simulink library "sfRobotExampleLib"  (R2025b)
settings: Solver=VariableStepAuto  StartTime=0.0  StopTime=10.0  RelTol=1e-3
undefined symbols (not defined in the file or in its folder): boxes, circles, dock
settings Model: Creator=The MathWorks, Inc.  LastModifiedBy=The MathWorks, Inc.
settings OptimizationCC: ReuseModelBlockBuffer=off
settings DebuggingCC: UnconnectedInputMsg=warning  UnconnectedOutputMsg=warning  UnconnectedLineMsg=warning
settings ModelReferenceCC: EnableRefExpFcnMdlSchedulingChecks=on
settings RTWCC: GPUComputeCapability=3.5  DLArmComputeVersion=19.05

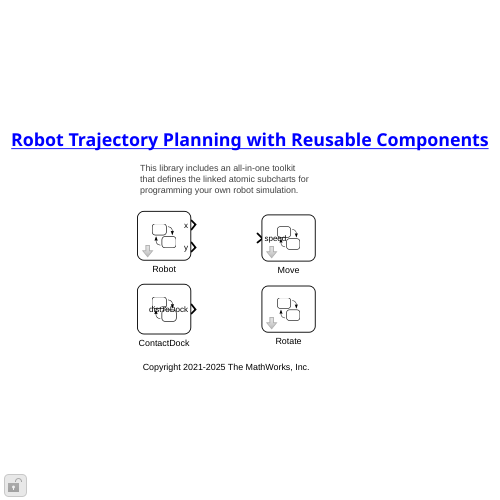
[thumbnail: Simulink's stored preview of the top-level diagram]
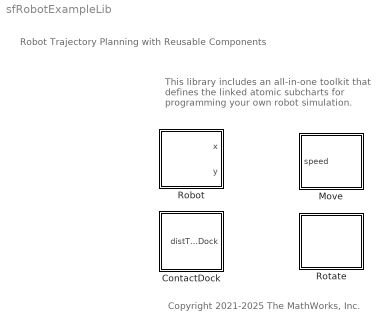
== system sfRobotExampleLib ==
  note: This library includes an all-in-one toolkit that defines the linked atomic subcharts for programming your own robot simulation.
  note: Copyright 2021-2025 The MathWorks, Inc.
  note: Robot Trajectory Planning with Reusable Components
  ContactDock : Stateflow chart  TreatAsAtomicUnit=on
  Move : Stateflow chart  TreatAsAtomicUnit=on  mask{stepsize=0}
      mask prompts: stepsize "Step size:"
  Robot : Stateflow chart  TreatAsAtomicUnit=on  mask{startPos=[0 0], startDir=3}
      mask prompts: startPos "Starting position (x,y)"; startDir "Starting direction (o'clock)"
  Rotate : Stateflow chart  TreatAsAtomicUnit=on  mask{angle=0}

== stateflow chart sfRobotExampleLib/Move ==
  state Forward
    Robot.move(stepsize);
    distance = distance + stepsize;
  state Backup
    Robot.move(-stepsize);
  (default) -> Forward
  Forward -> Backup [order 1] : [Robot.obstacle() == 1]
  Forward -> 13 [order 2] : [distance >= speed]
  Backup -> 20
  data: distance local =0; stepsize parameter; speed input

== stateflow chart sfRobotExampleLib/Rotate ==
  state Rotate
    Robot.rotate(direction*angle)
  25 -> Rotate : {direction=-1;}
  22 -> Rotate : {direction=1;}
  Rotate -> 13
  data: direction local; angle parameter

== stateflow chart sfRobotExampleLib/ContactDock ==
  state ContactDock
    distOld = distToDock;
    distToDock = Robot.distanceToDock();
  (default) -> ContactDock
  ContactDock -> 6 [order 1] : [distToDock >= distOld]
  ContactDock -> 7 [order 2]
  data: distToDock output =Inf; distOld local

== stateflow chart sfRobotExampleLib/Robot ==
  state INIT
    en:
    x = startPos(1); y = startPos(2);
    dx = cos((3-startDir)*pi/6); dy = sin((3-startDir)*pi/6);
  state dist = distanceToDock [function]
    (default) -> (junction 46) : {
        | dist = sqrt((x-dock(1))^2+(y-dock(2))^2);
        | }
  state move(speed) [function]
    (default) -> (junction 2) : {
        | x = x+speed*dx;
        | y = y+speed*dy;
        | }
  state rotate(angle) [function]
    (default) -> (junction 41) : {
        | c = cos(angle);
        | s = sin(angle);
        | M = [c -s; s c]*[dx;dy];
        | dx = M(1);
        | dy = M(2);
        | }
  state r = pointInCircle(circle) [function]
    (default) -> (junction 100)
    (junction 100) -> (junction 108) [order 1] : [(x-circle(1))^2+(y-circle(2))^2 > circle(3)^2]
    (junction 100) -> (junction 105) [order 2] : {r = true;}
    (junction 108) -> (junction 110) : {r = false;}
  state r = obstacle [function]
    (default) -> (junction 11) : {i = height(boxes);}
    (junction 11) -> (junction 74) [order 1] : [i>0]
    (junction 74) -> (junction 13) [order 1] : [pointInBox(boxes(i,:))]
    (junction 34) -> (junction 11)
    (junction 11) -> (junction 72) [order 2] : {i = height(circles);}
    (junction 74) -> (junction 34) [order 2] : {i = i-1;}
    (junction 13) -> (junction 84)
    (junction 72) -> (junction 89) [order 1] : [i>0]
    (junction 89) -> (junction 84) [order 1] : [pointInCircle(circles(i,:))]
    (junction 86) -> (junction 72)
    (junction 72) -> (junction 83) [order 2] : {r = false;}
    (junction 89) -> (junction 86) [order 2] : {i = i-1;}
    (junction 84) -> (junction 33) : {r=true;}
  state r = pointInBox(box) [function]
    (default) -> (junction 15)
    (junction 15) -> (junction 18) [order 1] : [x < box(1)]
    (junction 15) -> (junction 29) [order 2]
    (junction 18) -> (junction 63)
    (junction 29) -> (junction 63) [order 1] : [x > box(1)+box(3)]
    (junction 29) -> (junction 56) [order 2]
    (junction 63) -> (junction 64)
    (junction 56) -> (junction 64) [order 1] : [y > box(2)]
    (junction 56) -> (junction 59) [order 2]
    (junction 64) -> (junction 24)
    (junction 59) -> (junction 24) [order 1] : [y < box(2)-box(4)]
    (junction 59) -> (junction 62) [order 2] : {r = true;}
    (junction 24) -> (junction 65) : {r = false;}
  data: dist function_output double size=1; speed function_input double size=1; angle function_input double size=1; circle function_input double size=[1 3]; r function_output boolean size=1; r function_output boolean size=1; box function_input double size=[1 4]; r function_output boolean size=1; x output; y output; boxes parameter double; dx local; dy local; dock parameter double size=2; circles parameter; startPos parameter double size=2; startDir parameter double size=1
